simulink model "companion_io_ros2"  (R2026b)
undefined symbols (not defined in the file or in its folder): data, data_SL_Info, P, Ts
libraries: simulink x9, ros2lib x3, svdutilitieslib x2
settings Model: Creator=aomar  LastModifiedBy=aomar

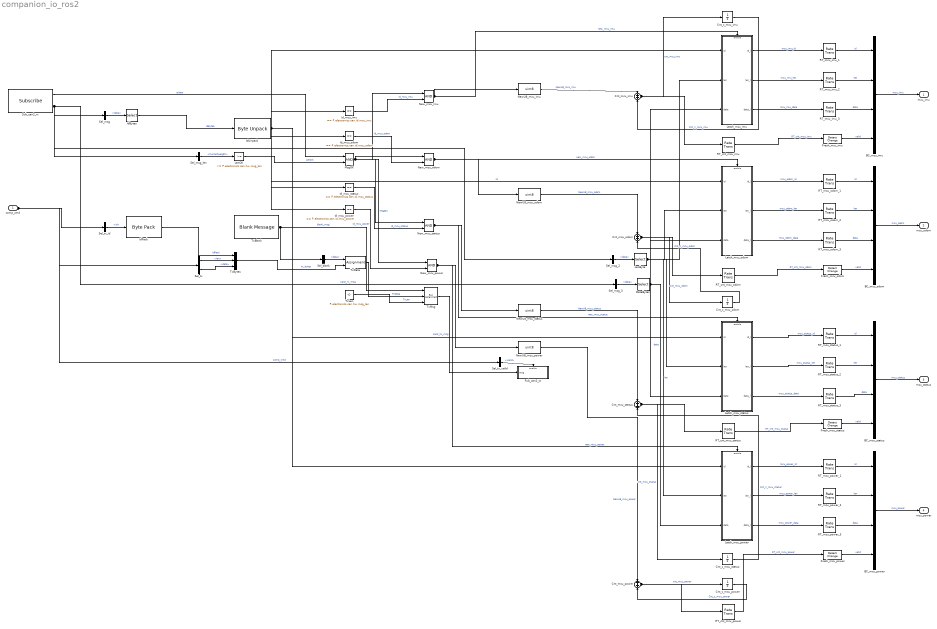
== system companion_io_ros2 ==
  comp_cmd : Inport  OutDataTypeStr=Bus: Bus_CanFrame64  SampleTime=Ts.comm  BusOutputAsStruct=on
  BC_mcu_imu : BusCreator  Inputs=4  OutDataTypeStr=Bus: Bus_CanFrame64  NonVirtualBus=on
      settings: InheritFromInputs=off
  BC_mcu_odom : BusCreator  Inputs=4  OutDataTypeStr=Bus: Bus_CanFrame64  NonVirtualBus=on
      settings: InheritFromInputs=off
  BC_mcu_power : BusCreator  Inputs=4  OutDataTypeStr=Bus: Bus_CanFrame64  NonVirtualBus=on
      settings: InheritFromInputs=off
  BC_mcu_status : BusCreator  Inputs=4  OutDataTypeStr=Bus: Bus_CanFrame64  NonVirtualBus=on
      settings: InheritFromInputs=off
  Cnt_mcu_imu : Sum  OutDataTypeStr=uint8
  Cnt_mcu_odom : Sum  OutDataTypeStr=uint8
  Cnt_mcu_power : Sum  OutDataTypeStr=uint8
  Cnt_mcu_status : Sum  OutDataTypeStr=uint8
  Cnt_z_mcu_imu : UnitDelay  SampleTime=Ts.base
  Cnt_z_mcu_odom : UnitDelay  SampleTime=Ts.base
  Cnt_z_mcu_power : UnitDelay  SampleTime=Ts.base
  Cnt_z_mcu_status : UnitDelay  SampleTime=Ts.base
  DataBytes : Selector  IndexOptions=Index vector (dialog)  Indices=6:69  OutputSizes=1
  Fresh_mcu_imu : simulink/Logic and Bit Operations/Detect Change  vinit=0  OutDataTypeStr=boolean
  Fresh_mcu_odom : simulink/Logic and Bit Operations/Detect Change  vinit=0  OutDataTypeStr=boolean
  Fresh_mcu_power : simulink/Logic and Bit Operations/Detect Change  vinit=0  OutDataTypeStr=boolean
  Fresh_mcu_status : simulink/Logic and Bit Operations/Detect Change  vinit=0  OutDataTypeStr=boolean
  IdBytes : Selector  IndexOptions=Index vector (dialog)  Indices=1:4  OutputSizes=1
  IdPack : svdutilitieslib/Byte Pack  maskPackedDataType=uint8  datatypes={'uint32'}  byteAlign=1  blockPlatform=arduinoert
      settings: LibrarySourceBlock=mcblib/Signal Management/Byte Pack
  IdUnpack : svdutilitieslib/Byte Unpack  dimensions={1}  datatypes={'uint32'}  byteAlign=1  blockPlatform=arduinoert
      settings: LibrarySourceBlock=mcblib/Signal Management/Byte Unpack
  Id_mcu_imu : simulink/Logic and Bit Operations/Compare To Constant  relop===  const=P.electronics.can.id.mcu_imu  OutDataTypeStr=boolean
  Id_mcu_odom : simulink/Logic and Bit Operations/Compare To Constant  relop===  const=P.electronics.can.id.mcu_odom  OutDataTypeStr=boolean
  Id_mcu_power : simulink/Logic and Bit Operations/Compare To Constant  relop===  const=P.electronics.can.id.mcu_power  OutDataTypeStr=boolean
  Id_mcu_status : simulink/Logic and Bit Operations/Compare To Constant  relop===  const=P.electronics.can.id.mcu_status  OutDataTypeStr=boolean
  Latch_mcu_imu : Subsystem  TreatAsAtomicUnit=on
  Latch_mcu_odom : Subsystem  TreatAsAtomicUnit=on
  Latch_mcu_power : Subsystem  TreatAsAtomicUnit=on
  Latch_mcu_status : Subsystem  TreatAsAtomicUnit=on
  LenByte : Selector  IndexOptions=Index vector (dialog)  Indices=5  OutputSizes=1
  LenOK : simulink/Logic and Bit Operations/Compare To Constant  relop=>=  const=P.electronics.can.hw.msg_len  OutDataTypeStr=boolean
  MsgOK : Logic  AllPortsSameDT=off  OutDataTypeStr=boolean
  NewU8_mcu_imu : DataTypeConversion  OutDataTypeStr=uint8  RndMeth=Nearest
  NewU8_mcu_odom : DataTypeConversion  OutDataTypeStr=uint8  RndMeth=Nearest
  NewU8_mcu_power : DataTypeConversion  OutDataTypeStr=uint8  RndMeth=Nearest
  NewU8_mcu_status : DataTypeConversion  OutDataTypeStr=uint8  RndMeth=Nearest
  New_mcu_imu : Logic  AllPortsSameDT=off  OutDataTypeStr=boolean
  New_mcu_odom : Logic  AllPortsSameDT=off  OutDataTypeStr=boolean
  New_mcu_power : Logic  AllPortsSameDT=off  OutDataTypeStr=boolean
  New_mcu_status : Logic  AllPortsSameDT=off  OutDataTypeStr=boolean
  Pub_can2_tx : Subsystem  TreatAsAtomicUnit=on
  RT_cnt_mcu_imu : RateTransition  OutPortSampleTime=Ts.imu
  RT_cnt_mcu_odom : RateTransition  OutPortSampleTime=Ts.ctrl
  RT_cnt_mcu_power : RateTransition  OutPortSampleTime=Ts.hk
  RT_cnt_mcu_status : RateTransition  OutPortSampleTime=Ts.comm
  RT_mcu_imu_1 : RateTransition  OutPortSampleTime=Ts.imu
  RT_mcu_imu_2 : RateTransition  OutPortSampleTime=Ts.imu
  RT_mcu_imu_3 : RateTransition  OutPortSampleTime=Ts.imu
  RT_mcu_odom_1 : RateTransition  OutPortSampleTime=Ts.ctrl
  RT_mcu_odom_2 : RateTransition  OutPortSampleTime=Ts.ctrl
  RT_mcu_odom_3 : RateTransition  OutPortSampleTime=Ts.ctrl
  RT_mcu_power_1 : RateTransition  OutPortSampleTime=Ts.hk
  RT_mcu_power_2 : RateTransition  OutPortSampleTime=Ts.hk
  RT_mcu_power_3 : RateTransition  OutPortSampleTime=Ts.hk
  RT_mcu_status_1 : RateTransition  OutPortSampleTime=Ts.comm
  RT_mcu_status_2 : RateTransition  OutPortSampleTime=Ts.comm
  RT_mcu_status_3 : RateTransition  OutPortSampleTime=Ts.comm
  Sel_blank : BusSelector  OutputSignals=data
  Sel_msg : BusSelector  OutputSignals=data
  Sel_msg_2 : BusSelector  OutputSignals=data
  Sel_msg_3 : BusSelector  OutputSignals=data
  Sel_msg_len : BusSelector  OutputSignals=data_SL_Info.CurrentLength
  Sel_tx : BusSelector  OutputSignals=len,data
  Sel_tx_id : BusSelector  OutputSignals=id
  Sel_tx_valid : BusSelector  OutputSignals=valid
  Sub_can2_rx : ros2lib/Subscribe  topicSource=Specify your own  topic=/can2/rx  messageType=std_msgs/UInt8MultiArray  SubscriberMode=At sample time  sampleTime=Ts.base  CallbackGroupType=Default  CallbackGroupName=callback_group_1  QOSHistory=Keep last  QOSDepth=16  QOSReliability=Reliable  QOSDurability=Volatile  QOSDeadline=Inf  QOSLifespan=Inf  QOSLiveliness=Automatic  QOSLeaseDuration=Inf  QOSAvoidROSNamespaceConventions=off
  TxBlank : ros2lib/Blank Message  messageClass=Message  entityType=std_msgs/UInt8MultiArray  messageType=std_msgs/UInt8MultiArray  SampleTime=Ts.comm
  TxBytes : Concatenate  NumInputs=3
  TxData : Assignment  DiagnosticForDimensions=Warning  IndexOptions=Index vector (dialog)  Indices=1:P.electronics.can.hw.msg_len  OutputSizes=1
  TxLen : Constant  Value=P.electronics.can.hw.msg_len  OutDataTypeStr=uint32  SampleTime=Ts.comm
  TxMsg : BusAssignment  AssignedSignals=data,data_SL_Info.CurrentLength
  mcu_imu : Outport  OutDataTypeStr=Bus: Bus_CanFrame64  SampleTime=Ts.imu  BusOutputAsStruct=on
  mcu_odom : Outport  Port=2  OutDataTypeStr=Bus: Bus_CanFrame64  SampleTime=Ts.ctrl  BusOutputAsStruct=on
  mcu_status : Outport  Port=3  OutDataTypeStr=Bus: Bus_CanFrame64  SampleTime=Ts.comm  BusOutputAsStruct=on
  mcu_power : Outport  Port=4  OutDataTypeStr=Bus: Bus_CanFrame64  SampleTime=Ts.hk  BusOutputAsStruct=on
  wires:
  comp_cmd/1 -> Sel_tx_valid/1, Sel_tx/1, Sel_tx_id/1  "comp_cmd"
  Sub_can2_rx/1 -> MsgOK/1  "IsNew"
  Sub_can2_rx/2 -> Sel_msg_3/1, Sel_msg_2/1, Sel_msg_len/1, Sel_msg/1  "can2_rx_msg"
  Sel_msg/1 -> IdBytes/1  "<data>"
  Sel_tx_id/1 -> IdPack/1  "<id>"
  IdBytes/1 -> IdUnpack/1  "IdBytes"
  IdPack/1 -> TxBytes/1  "IdPack"
  Sel_msg_len/1 -> LenOK/1  "<CurrentLength>"
  Sel_tx/1 -> TxBytes/2  "<len>"
  Sel_tx/2 -> TxBytes/3  "<data>"
  TxBytes/1 -> TxData/2  "tx_bytes"
  LenOK/1 -> MsgOK/2  "LenOK"
  IdUnpack/1 -> Latch_mcu_power/1(id), Latch_mcu_status/1(id), Id_mcu_power/1, Latch_mcu_imu/1(id), Id_mcu_status/1, Latch_mcu_odom/1(id), Id_mcu_imu/1, Id_mcu_odom/1  "id"
  TxBlank/1 -> TxMsg/1, Sel_blank/1  "blank_msg"
  Sel_blank/1 -> TxData/1  "<data>"
  Id_mcu_imu/1 -> New_mcu_imu/2  "Id_mcu_imu"
  Id_mcu_odom/1 -> New_mcu_odom/2  "Id_mcu_odom"
  MsgOK/1 -> New_mcu_power/1, New_mcu_imu/1, New_mcu_status/1, New_mcu_odom/1  "MsgOK"
  Id_mcu_status/1 -> New_mcu_status/2  "Id_mcu_status"
  Id_mcu_power/1 -> New_mcu_power/2  "Id_mcu_power"
  TxLen/1 -> TxMsg/3  "TxLen"
  TxData/1 -> TxMsg/2  "TxData"
  New_mcu_imu/1 -> Latch_mcu_imu/Enable, NewU8_mcu_imu/1  "new_mcu_imu"
  New_mcu_odom/1 -> NewU8_mcu_odom/1, Latch_mcu_odom/Enable  "new_mcu_odom"
  New_mcu_status/1 -> Latch_mcu_status/Enable, NewU8_mcu_status/1  "new_mcu_status"
  New_mcu_power/1 -> Latch_mcu_power/Enable, NewU8_mcu_power/1  "new_mcu_power"
  TxMsg/1 -> Pub_can2_tx/1(msg)  "can2_tx_msg"
  Sel_tx_valid/1 -> Pub_can2_tx/Enable  "<valid>"
  NewU8_mcu_imu/1 -> Cnt_mcu_imu/1  "NewU8_mcu_imu"
  NewU8_mcu_odom/1 -> Cnt_mcu_odom/1  "NewU8_mcu_odom"
  NewU8_mcu_status/1 -> Cnt_mcu_status/1  "NewU8_mcu_status"
  NewU8_mcu_power/1 -> Cnt_mcu_power/1  "NewU8_mcu_power"
  Sel_msg_2/1 -> LenByte/1  "<data>"
  Sel_msg_3/1 -> DataBytes/1  "<data>"
  Cnt_mcu_imu/1 -> Cnt_z_mcu_imu/1, RT_cnt_mcu_imu/1  "cnt_mcu_imu"
  Cnt_mcu_odom/1 -> Cnt_z_mcu_odom/1, RT_cnt_mcu_odom/1  "cnt_mcu_odom"
  Cnt_mcu_status/1 -> Cnt_z_mcu_status/1, RT_cnt_mcu_status/1  "cnt_mcu_status"
  Cnt_mcu_power/1 -> RT_cnt_mcu_power/1, Cnt_z_mcu_power/1  "cnt_mcu_power"
  LenByte/1 -> Latch_mcu_power/2(len), Latch_mcu_imu/2(len), Latch_mcu_status/2(len), Latch_mcu_odom/2(len)  "len"
  DataBytes/1 -> Latch_mcu_power/3(data), Latch_mcu_imu/3(data), Latch_mcu_status/3(data), Latch_mcu_odom/3(data)  "data"
  Cnt_z_mcu_imu/1 -> Cnt_mcu_imu/2  "Cnt_z_mcu_imu"
  Cnt_z_mcu_odom/1 -> Cnt_mcu_odom/2  "Cnt_z_mcu_odom"
  Cnt_z_mcu_status/1 -> Cnt_mcu_status/2  "Cnt_z_mcu_status"
  Cnt_z_mcu_power/1 -> Cnt_mcu_power/2  "Cnt_z_mcu_power"
  RT_cnt_mcu_imu/1 -> Fresh_mcu_imu/1  "RT_cnt_mcu_imu"
  RT_cnt_mcu_odom/1 -> Fresh_mcu_odom/1  "RT_cnt_mcu_odom"
  RT_cnt_mcu_status/1 -> Fresh_mcu_status/1  "RT_cnt_mcu_status"
  RT_cnt_mcu_power/1 -> Fresh_mcu_power/1  "RT_cnt_mcu_power"
  Latch_mcu_imu/1(id_l) -> RT_mcu_imu_1/1  "mcu_imu_id"
  Latch_mcu_imu/2(len_l) -> RT_mcu_imu_2/1  "mcu_imu_len"
  Latch_mcu_imu/3(data_l) -> RT_mcu_imu_3/1  "mcu_imu_data"
  Latch_mcu_odom/1(id_l) -> RT_mcu_odom_1/1  "mcu_odom_id"
  Latch_mcu_odom/2(len_l) -> RT_mcu_odom_2/1  "mcu_odom_len"
  Latch_mcu_odom/3(data_l) -> RT_mcu_odom_3/1  "mcu_odom_data"
  Latch_mcu_status/1(id_l) -> RT_mcu_status_1/1  "mcu_status_id"
  Latch_mcu_status/2(len_l) -> RT_mcu_status_2/1  "mcu_status_len"
  Latch_mcu_status/3(data_l) -> RT_mcu_status_3/1  "mcu_status_data"
  Latch_mcu_power/1(id_l) -> RT_mcu_power_1/1  "mcu_power_id"
  Latch_mcu_power/2(len_l) -> RT_mcu_power_2/1  "mcu_power_len"
  Latch_mcu_power/3(data_l) -> RT_mcu_power_3/1  "mcu_power_data"
  RT_mcu_imu_1/1 -> BC_mcu_imu/1  "id"
  RT_mcu_imu_2/1 -> BC_mcu_imu/2  "len"
  RT_mcu_imu_3/1 -> BC_mcu_imu/3  "data"
  RT_mcu_odom_1/1 -> BC_mcu_odom/1  "id"
  RT_mcu_odom_2/1 -> BC_mcu_odom/2  "len"
  RT_mcu_odom_3/1 -> BC_mcu_odom/3  "data"
  RT_mcu_status_1/1 -> BC_mcu_status/1  "id"
  RT_mcu_status_2/1 -> BC_mcu_status/2  "len"
  RT_mcu_status_3/1 -> BC_mcu_status/3  "data"
  RT_mcu_power_1/1 -> BC_mcu_power/1  "id"
  RT_mcu_power_2/1 -> BC_mcu_power/2  "len"
  RT_mcu_power_3/1 -> BC_mcu_power/3  "data"
  Fresh_mcu_imu/1 -> BC_mcu_imu/4  "valid"
  Fresh_mcu_odom/1 -> BC_mcu_odom/4  "valid"
  Fresh_mcu_status/1 -> BC_mcu_status/4  "valid"
  Fresh_mcu_power/1 -> BC_mcu_power/4  "valid"
  BC_mcu_imu/1 -> mcu_imu/1  "mcu_imu"
  BC_mcu_odom/1 -> mcu_odom/1  "mcu_odom"
  BC_mcu_status/1 -> mcu_status/1  "mcu_status"
  BC_mcu_power/1 -> mcu_power/1  "mcu_power"

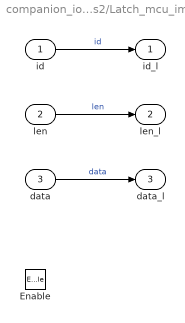
== system companion_io_ros2/Latch_mcu_imu ==
  id : Inport
  len : Inport  Port=2
  data : Inport  Port=3
  Enable : EnablePort
  id_l : Outport  InitialOutput=0
  len_l : Outport  Port=2  InitialOutput=0
  data_l : Outport  Port=3  InitialOutput=0
  wires:
  id/1 -> id_l/1  "id"
  len/1 -> len_l/1  "len"
  data/1 -> data_l/1  "data"

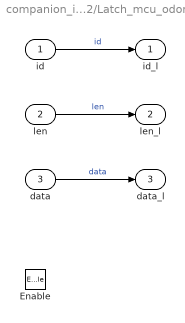
== system companion_io_ros2/Latch_mcu_odom ==
  id : Inport
  len : Inport  Port=2
  data : Inport  Port=3
  Enable : EnablePort
  id_l : Outport  InitialOutput=0
  len_l : Outport  Port=2  InitialOutput=0
  data_l : Outport  Port=3  InitialOutput=0
  wires:
  id/1 -> id_l/1  "id"
  len/1 -> len_l/1  "len"
  data/1 -> data_l/1  "data"

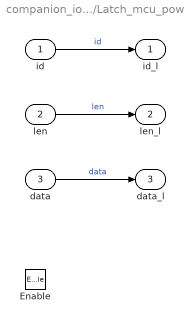
== system companion_io_ros2/Latch_mcu_power ==
  id : Inport
  len : Inport  Port=2
  data : Inport  Port=3
  Enable : EnablePort
  id_l : Outport  InitialOutput=0
  len_l : Outport  Port=2  InitialOutput=0
  data_l : Outport  Port=3  InitialOutput=0
  wires:
  id/1 -> id_l/1  "id"
  len/1 -> len_l/1  "len"
  data/1 -> data_l/1  "data"

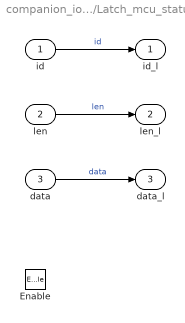
== system companion_io_ros2/Latch_mcu_status ==
  id : Inport
  len : Inport  Port=2
  data : Inport  Port=3
  Enable : EnablePort
  id_l : Outport  InitialOutput=0
  len_l : Outport  Port=2  InitialOutput=0
  data_l : Outport  Port=3  InitialOutput=0
  wires:
  id/1 -> id_l/1  "id"
  len/1 -> len_l/1  "len"
  data/1 -> data_l/1  "data"

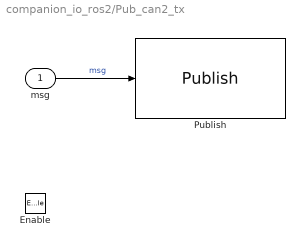
== system companion_io_ros2/Pub_can2_tx ==
  msg : Inport
  Enable : EnablePort
  Publish : ros2lib/Publish  topicSource=Specify your own  topic=/can2/tx  messageType=std_msgs/UInt8MultiArray  QOSHistory=Keep last  QOSDepth=16  QOSReliability=Reliable  QOSDurability=Volatile  QOSDeadline=Inf  QOSLifespan=Inf  QOSLiveliness=Automatic  QOSLeaseDuration=Inf  QOSAvoidROSNamespaceConventions=off
  wires:
  msg/1 -> Publish/1  "msg"
